simulink model "ARDroneReplay_BatistaKF"  (R2026a)
settings: Solver=ode1  StopTime=30  FixedStep=0.005
model workspace (MAT data in the model file):
  P0 = [1  0  0  0  0  0; 0  1  0  0  0  0; 0  0  1  0  0  0; 0  0  0  0.01  0  0; 0  0  0  0  0.01  0; 0  0  0  0  0  0.01]
  Th = [0.0245  0  0; 0  0.0245  0; 0  0  0.0245]
  Xi = [0.0005894461125  0  0  0  0  0; 0  0.0005894461125  0  0  0  0; 0  0  0.0005894461125  0  0  0; 0  0  0  1e-05  0  0; 0  0  0  0  1e-05  0; 0  0  0  0  0  1e-05]
  acc_cal_T = 0
  b_art_degps = [0 0 0]
  x0 = [0; 0; -9.81; 0; 0; 0]
libraries: ARBlocks x1
settings Model: PacingRate=5

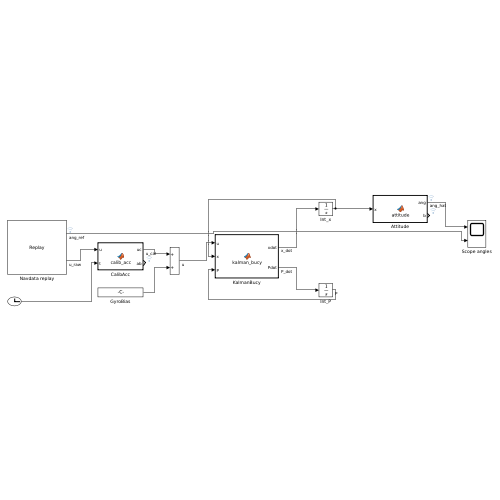
[thumbnail: Simulink's stored preview of the top-level diagram]
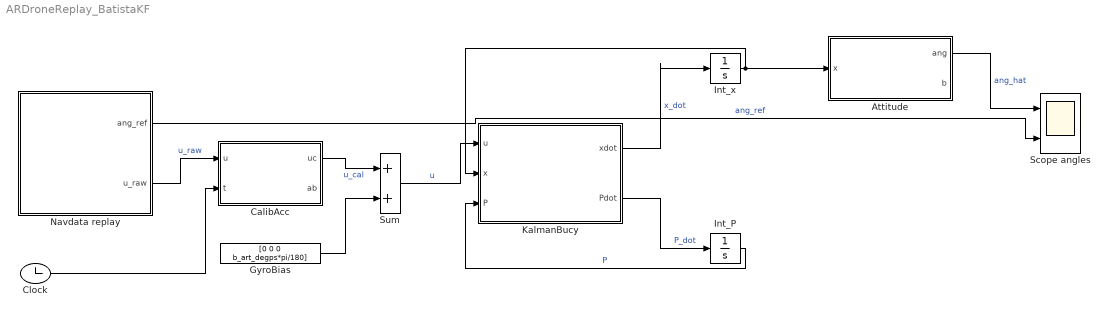
== system ARDroneReplay_BatistaKF ==
  Attitude : MATLAB Function  TreatAsAtomicUnit=on
  CalibAcc : MATLAB Function  TreatAsAtomicUnit=on
  Clock : Clock
  GyroBias : Constant  Value=[0 0 0 b_art_degps*pi/180]
  Int_P : Integrator  InitialCondition=P0
  Int_x : Integrator  InitialCondition=x0
  KalmanBucy : MATLAB Function  TreatAsAtomicUnit=on
  Navdata replay : Subsystem
      mask Display: disp('Replay')
  Scope angles : Scope  NumInputPorts=2
      settings: YLabel=Roll, pitch [deg]: KF (1) vs onboard (2)
  Sum : Sum
  wires:
  Navdata replay/2(u_raw) -> CalibAcc/1(u)  "u_raw"
  Clock/1 -> CalibAcc/2(t)
  CalibAcc/1(uc) -> Sum/1  "u_cal"
  GyroBias/1 -> Sum/2
  KalmanBucy/1(xdot) -> Int_x/1  "x_dot"
  KalmanBucy/2(Pdot) -> Int_P/1  "P_dot"
  Int_x/1 -> KalmanBucy/2(x), Attitude/1(x)
  Int_P/1 -> KalmanBucy/3(P)  "P"
  Sum/1 -> KalmanBucy/1(u)  "u"
  Attitude/1(ang) -> Scope angles/1  "ang_hat"
  Navdata replay/1(ang_ref) -> Scope angles/2  "ang_ref"

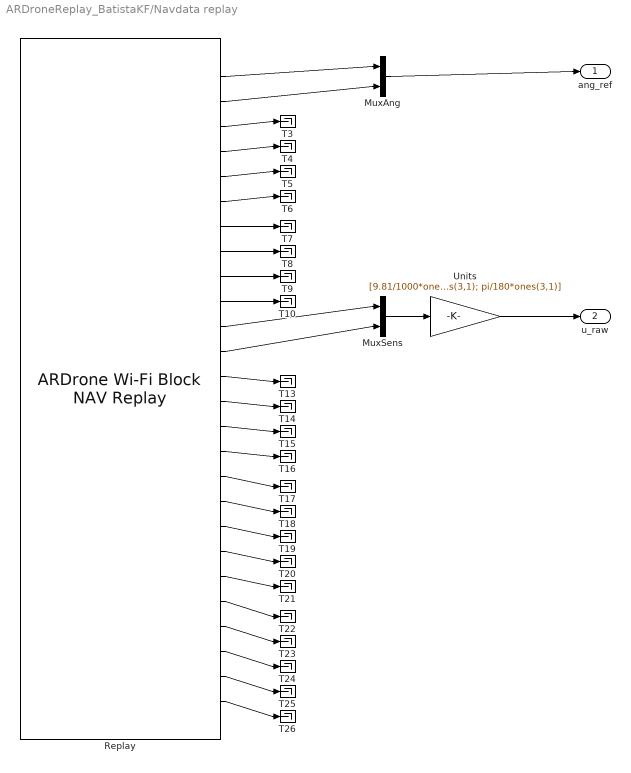
== system ARDroneReplay_BatistaKF/Navdata replay ==
  MuxAng : Mux  Inputs=2
  MuxSens : Mux  Inputs=2
  Replay : ARBlocks/ARDrone Wi-Fi  Block NAV Replay  SystemSampleTime=-1  VariantActivationTime=update diagram  EmptyChoice=off  PassThrough=off  PassThroughVariantControl=(default)  EmptyChoiceVariantControl=(default)  AllowFlexibleInterface=on  Latency=0  AutoFrameSizeCalculation=off
  T{3..10,13..26} (22 alike) : Terminator
  Units : Gain  Gain=[9.81/1000*ones(3,1); pi/180*ones(3,1)]
  ang_ref : Outport
  u_raw : Outport  Port=2
  wires:
  Replay/3 -> T3/1
  Replay/4 -> T4/1
  Replay/5 -> T5/1
  Replay/6 -> T6/1
  Replay/7 -> T7/1
  Replay/8 -> T8/1
  Replay/9 -> T9/1
  Replay/10 -> T10/1
  Replay/13 -> T13/1
  Replay/14 -> T14/1
  Replay/15 -> T15/1
  Replay/16 -> T16/1
  Replay/17 -> T17/1
  Replay/18 -> T18/1
  Replay/19 -> T19/1
  Replay/20 -> T20/1
  Replay/21 -> T21/1
  Replay/22 -> T22/1
  Replay/23 -> T23/1
  Replay/24 -> T24/1
  Replay/25 -> T25/1
  Replay/26 -> T26/1
  Replay/1 -> MuxAng/1
  Replay/2 -> MuxAng/2
  Replay/11 -> MuxSens/1
  Replay/12 -> MuxSens/2
  MuxAng/1 -> ang_ref/1
  MuxSens/1 -> Units/1
  Units/1 -> u_raw/1

== matlab function ARDroneReplay_BatistaKF/KalmanBucy ==
  data: u input; xdot output; x input; P input; Pdot output; Xi parameter; Th parameter
function [xdot, Pdot] = kalman_bucy(u, x, P, Xi, Th)
% Continuous-time Kalman filter for the Batista et al. system (2)/(10).
% u = [accelerometer (m/s^2); rate gyro (rad/s)], x = [x1; bias], P: 6x6.
y = u(1:3);  w = u(4:6);
Sw = [0 -w(3) w(2); w(3) 0 -w(1); -w(2) w(1) 0];
Sy = [0 -y(3) y(2); y(3) 0 -y(1); -y(2) y(1) 0];
A  = [-Sw -Sy; zeros(3) zeros(3)];
C  = [eye(3) zeros(3)];
K  = P*C' / Th;
xdot = A*x + K*(y - C*x);
Pdot = A*P + P*A' + Xi - K*(C*P);
end

== matlab function ARDroneReplay_BatistaKF/CalibAcc ==
  settings: updateMethod=DISCRETE  sampleTime=0.005
  data: u input; uc output; t input; ab output; acc_cal_T parameter
function [uc, ab] = calib_acc(u, t, acc_cal_T)
% Level-on-the-ground calibration of the accelerometer (ax, ay), causal.
% Running mean over t in [0.05, acc_cal_T], frozen afterwards. acc_cal_T = 0: off.
persistent s n
if isempty(s), s = zeros(2,1); n = 0; end
if acc_cal_T > 0 && t < acc_cal_T && t >= 0.05
    s = s + u(1:2);  n = n + 1;
end
ab = zeros(6,1);
if acc_cal_T > 0 && n > 0, ab(1:2) = s/n; end
uc = u - ab;
end

== matlab function ARDroneReplay_BatistaKF/Attitude ==
  data: x input; ang output; b output
function [ang, b] = attitude(x)
% Roll/pitch [deg] from the filtered body-frame vector (sensor convention
% az = -g at rest) and gyro bias estimate [deg/s].
x1 = x(1:3);
n  = norm(x1);
phi = atan2(-x1(2), -x1(3))*180/pi;
if n > eps
    theta = asin(x1(1)/n)*180/pi;
else
    theta = 0;
end
ang = [phi; theta];
b = x(4:6)*180/pi;
end
